simulink model "ASM_Traffic_MultiCore"  (R2026a)
settings: Solver=ode1  StartTime=SIM.tstart.v  StopTime=SIM.tend.v  FixedStep=SIM.StepSize.v
PostLoadFcn:
  | if any(exist('dsrtsu_mdlpostloadfcn', 'file') ~= 0), dsrtsu_mdlpostloadfcn('Execute', bdroot); end
  | try, asm_mdl_postloadfcn(bdroot, 'UpdateModel', 3600); catch, disp(lasterr); end,
InitFcn:
  | , if any(exist('rtifpga_mdlclblib', 'file') ~= 0), rtifpga_mdlclblib('Init', bdroot); end,
  | , if any(exist('dsmpb_private', 'file') ~= 0), dsmpb_private('dsmpb_mdlclblib', 'Init', bdroot); end,
model workspace (MAT data in the model file):
  asmReferencePath = [0 0.01 0.02 0.03 0.04 0.05 0.06 0.07 0.08 0.09 0.1 0.11 ... (350007 elements, 50001x7)]
  roadBounds : Simulink.Parameter (value not decoded)
  safetyAxes : Simulink.Parameter (value not decoded)
undefined symbols (not defined in the file): _to_, a0b2, ASM_BrakeHydraulics_DemoSystems, ASM_VehicleDynamics_DemoSystems, b98103fe8ad365046cd0, BrakeCircuit, controllerConfig, CPT, Crankshaft, DiscIntNeverNeededParam, dsmsi, FinalDriveAssembly, MDL, ModeSignals, mu, Pos_BrakePedal_Maneuver, rad, RefSignals, roadFamilyData, roadFamilyId, s_to_rpm, SIM, SoftECU, Suspension, Tire, Transmission
libraries: ASM_Traffic_lib x135, simulink x98, ASM_Utils_lib x77, ASM_VehicleDynamics_lib x70, ASM_Environment_lib x22, dsmpblib x20, dsmsilib x15, MDLD_Utils_lib x10, ASM_BrakeHydraulics_lib x3, sl_discontinuities x2
(part 9 of 65)

== system ASM_Traffic_MultiCore/AnimationInterface/ANIMATION_INTERFACE/Lane_Sensor ==
  Environment_Animation : Inport
  Bus Selector1 : BusSelector  OutputSignals=Pos_Left[x;y;z][m],Yaw_Angle_Left[deg],MarkerType_Left[],Pos_Right[x;y;z][m],Yaw_Angle_Right[deg],MarkerType_Right[]
  Enable_Data_Transfer : Constant
  LaneSensor : dsmsilib/dsmsi_simulation_data_objects_BL1  Priority=10001  parameterStr="{\"Version\":1,\"TransformInput\":false,\"EnableInput\":true,\"Objects\":[{\"Name\":\"LaneSensor_Left\",\"TypeClass\":{\"Name\":\"Transformation\",\"Class\":1,\"SignalProperty\":null,\"TransformationProperty\":{\"TransformMatrixIn\":false,\"TransformMatrixOut\":false,\"AngleInterpretation\":0,\"TransformationOrder\":0,\"RotationOrder\":0,\"TranslationAsParameter\":false,\"Translation\":\"[0 0 0]\",\"RotationAsParameter\":false,\"Rotation\":\"[0 0 0]\",\"ScalingAsParameter\":false,\"Scaling\":\"[1 1 1]\",\"ObjectsCount\":1},\"PositionAndScaleProperty\":null,\"PositionProperty\":null},\"Children\":[],\"Oid\":1},{\"Name\":\"LaneSensor_Right\",\"TypeClass\":{\"Name\":\"Transformation\",\"Class\":1,\"SignalProperty\":null,\"TransformationProperty\":{\"TransformMatrixIn\":false,\"TransformMatrixOut\":false,\"AngleInterpretation\":0,\"TransformationOrder\":0,\"RotationOrder\":0,\"TranslationAsParameter\":false,\"Translation\":\"[0 0 0]\",\"RotationAsParameter\":false,\"Rotation\":\"[0 0 0]\",\"ScalingAsParameter\":false,\"Scaling\":\"[1 1 1]\",\"ObjectsCount\":1},\"PositionAndScaleProperty\":null,\"PositionProperty\":null},\"Children\":[],\"Oid\":2}]}"  evalStr=dsmsi(gcb, 'EvalJson')  sampleTime=-1  globalBlockId=0  objectsBlockId=dsmsi(gcb, 'GetObjectBlockId')  objectsBlockGuiOpen=dsmsi(gcb, 'GetSdoGuiStatus')  dialogIsOpen=0  blockVersion=60  highPrecision=0  validNameBckp=LaneSensor
      settings: SourceProductName=dSPACE MSI Blockset
  Sensor_L_Rotation : Subsystem
  Sensor_L_Scaling : Subsystem
  Sensor_L_Translation : Subsystem
  Sensor_R_Rotation : Subsystem
  Sensor_R_Scaling : Subsystem
  Sensor_R_Translation : Subsystem
  Sw_Pitch_Angle_Offset_For_AURELION[0|1] : Constant
  wires:
  Sw_Pitch_Angle_Offset_For_AURELION[0|1]/1 -> Sensor_L_Rotation/1(Sw_Pitch_Angle_Offset), Sensor_R_Rotation/1(Sw_Pitch_Angle_Offset)
  Bus Selector1/5 -> Sensor_R_Rotation/2(In)  "<Yaw_Angle_Right[deg]>"
  Sensor_R_Rotation/1(Out) -> LaneSensor/6
  Enable_Data_Transfer/1 -> LaneSensor/1
  Sensor_R_Scaling/1(Out) -> LaneSensor/7
  Sensor_L_Scaling/1(Out) -> LaneSensor/4
  Bus Selector1/3 -> Sensor_L_Scaling/1(In)  "<MarkerType_Left[]>"
  Sensor_L_Rotation/1(Out) -> LaneSensor/3
  Bus Selector1/2 -> Sensor_L_Rotation/2(In)  "<Yaw_Angle_Left[deg]>"
  Sensor_R_Translation/1(Out) -> LaneSensor/5
  Sensor_L_Translation/1(Out) -> LaneSensor/2
  Bus Selector1/1 -> Sensor_L_Translation/1(In)  "<Pos_Left[x;y;z][m]>"
  Bus Selector1/6 -> Sensor_R_Scaling/1(In)  "<MarkerType_Right[]>"
  Bus Selector1/4 -> Sensor_R_Translation/1(In)  "<Pos_Right[x;y;z][m]>"
  Environment_Animation/1 -> Bus Selector1/1

== system ASM_Traffic_MultiCore/AnimationInterface/ANIMATION_INTERFACE/Lane_Sensor_Dynamic_Instruments ==
  Environment_Animation : Inport
  Bus Selector3 : BusSelector  OutputSignals=Network_Item_Type_Veh[],Distance_MeasPnt_Marker_Left[m],Distance_MeasPnt_Marker_Right[m],Velocity_MeasPnt_Marker_Left[m|s],Velocity_MeasPnt_Marker_Right[m|s]
  CalcLDWState : Subsystem
  Enable_Data_Transfer : Constant
  LaneSensor_Dynamic_Instruments : dsmsilib/dsmsi_simulation_data_objects_BL1  Priority=10001  parameterStr="{\"Version\":1,\"TransformInput\":false,\"EnableInput\":true,\"Objects\":[{\"Name\":\"LDWState_L[]\",\"TypeClass\":{\"Name\":\"Signal\",\"Class\":3,\"SignalProperty\":{\"Description\":null,\"Unit\":null,\"Type\":0,\"Length\":1,\"ObjectsCount\":1},\"TransformationProperty\":null,\"PositionAndScaleProperty\":null,\"PositionProperty\":null},\"Children\":[],\"Oid\":1},{\"Name\":\"LDWState_R[]\",\"TypeClass\":{\"Name\":\"Signal\",\"Class\":3,\"SignalProperty\":{\"Description\":null,\"Unit\":null,\"Type\":0,\"Length\":1,\"ObjectsCount\":1},\"TransformationProperty\":null,\"PositionAndScaleProperty\":null,\"PositionProperty\":null},\"Children\":[],\"Oid\":2},{\"Name\":\"LatDistance Left\",\"TypeClass\":{\"Name\":\"Signal\",\"Class\":3,\"SignalProperty\":{\"Description\":null,\"Unit\":\"m\",\"Type\":0,\"Length\":1,\"ObjectsCount\":1},\"TransformationProperty\":null,\"PositionAndScaleProperty\":null,\"PositionProperty\":null},\"Children\":[],\"Oid\":3},{\"Name\":\"LatDistance Right\",\"TypeClass\":{\"Name\":\"Signal\",\"Class\":3,\"SignalProperty\":{\"Description\":null,\"Unit\":\"m\",\"Type\":0,\"Length\":1,\"ObjectsCount\":1},\"TransformationProperty\":null,\"PositionAndScaleProperty\":null,\"PositionProperty\":null},\"Children\":[],\"Oid\":4},{\"Name\":\"LatVelocity Left\",\"TypeClass\":{\"Name\":\"Signal\",\"Class\":3,\"SignalProperty\":{\"Description\":null,\"Unit\":\"m/s\",\"Type\":0,\"Length\":1,\"ObjectsCount\":1},\"TransformationProperty\":null,\"PositionAndScaleProperty\":null,\"PositionProperty\":null},\"Children\":[],\"Oid\":5},{\"Name\":\"LatVelocity Right\",\"TypeClass\":{\"Name\":\"Signal\",\"Class\":3,\"SignalProperty\":{\"Description\":null,\"Unit\":\"m/s\",\"Type\":0,\"Length\":1,\"ObjectsCount\":1},\"TransformationProperty\":null,\"PositionAndScaleProperty\":null,\"PositionProperty\":null},\"Children\":[],\"Oid\":6}]}"  evalStr=dsmsi(gcb, 'EvalJson')  sampleTime=-1  globalBlockId=0  objectsBlockId=dsmsi(gcb, 'GetObjectBlockId')  objectsBlockGuiOpen=dsmsi(gcb, 'GetSdoGuiStatus')  dialogIsOpen=0  blockVersion=60  highPrecision=0  validNameBckp=LaneSensor_Dynamic_Instruments
      settings: SourceProductName=dSPACE MSI Blockset
  Selector1 : Selector  IndexOptions=Index vector (dialog)  Indices=[1]  OutputSizes=1
  Selector2 : Selector  IndexOptions=Index vector (dialog)  Indices=[2]  OutputSizes=1
  Selector3 : Selector  IndexOptions=Index vector (dialog)  Indices=[1]  OutputSizes=1
  Selector4 : Selector  IndexOptions=Index vector (dialog)  Indices=[2]  OutputSizes=1
  wires:
  Enable_Data_Transfer/1 -> LaneSensor_Dynamic_Instruments/1
  Environment_Animation/1 -> Bus Selector3/1
  Bus Selector3/3 -> Selector2/1  "<Distance_MeasPnt_Marker_Right[m]>"
  Bus Selector3/1 -> CalcLDWState/1(NetworkItemType[])  "<Network_Item_Type_Veh[]>"
  Bus Selector3/2 -> Selector1/1  "<Distance_MeasPnt_Marker_Left[m]>"
  Bus Selector3/5 -> Selector4/1  "<Velocity_MeasPnt_Marker_Right[m|s]>"
  CalcLDWState/1(LDWState_L[]) -> LaneSensor_Dynamic_Instruments/2
  Selector2/1 -> LaneSensor_Dynamic_Instruments/5, CalcLDWState/3(Dist_R[m])
  Selector1/1 -> LaneSensor_Dynamic_Instruments/4, CalcLDWState/2(Dist_L[m])
  Bus Selector3/4 -> Selector3/1  "<Velocity_MeasPnt_Marker_Left[m|s]>"
  Selector3/1 -> LaneSensor_Dynamic_Instruments/6
  Selector4/1 -> LaneSensor_Dynamic_Instruments/7
  CalcLDWState/2(LDWState_R[]) -> LaneSensor_Dynamic_Instruments/3

== system ASM_Traffic_MultiCore/AnimationInterface/ANIMATION_INTERFACE/Sensors ==
  Transform_In : Inport
  Sw_Sensor_Selector[] : Inport  Port=2
  Sw_Sensor_Animation[] : Inport  Port=3
  Environment_Animation : Inport  Port=4
  Bus Selector1 : BusSelector  OutputSignals=ObjectSensor2D_1,ObjectSensor2D_2,ObjectSensor2D_3,ObjectSensor2D_4,ObjectSensor2D_5,ObjectSensor2D_6,ObjectSensor2D_7
  Bus Selector2 : BusSelector  OutputSignals=Line_Sensor.Pos_Road_Lane_Animation_CoorSys_E,Line_Sensor.Pos_Road_Shape_Line_Animation_CoorSys_E,Line_Sensor.Pos_Road_Shape_ContObj_Animation_CoorSys_E,Line_Sensor.Pos_Junction_Border_Animation_CoorSys_E,Line_Sensor.Pos_Junction_Shape_Line_Animation_CoorSys_E,Line_Sensor.Pos_Junction_Shape_ContObj_Animation_CoorSys_E
  Bus Selector3 : BusSelector  OutputSignals=ObjectSensor3D_1,ObjectSensor3D_2,ObjectSensor3D_3
  Bus Selector4 : BusSelector  OutputSignals=TrafficSign_Sensor_Dyn
  Bus Selector5 : BusSelector  OutputSignals=ObjectSensor3D_1_RadarEffects,ObjectSensor3D_2_RadarEffects,ObjectSensor3D_3_RadarEffects
  Bus Selector6 : BusSelector  OutputSignals=ObjectSensor3D_1_CustomPoints,ObjectSensor3D_2_CustomPoints,ObjectSensor3D_3_CustomPoints
  Enable_Data_Transfer : Constant
  Line_Sensor_Junction_Border_Points : Subsystem
  Line_Sensor_Junction_Shape_ContObj_Points : Subsystem
  Line_Sensor_Junction_Shape_Line_Points : Subsystem
  Line_Sensor_Road_Lane_Points : Subsystem
  Line_Sensor_Road_Shape_ContObj_Points : Subsystem
  Line_Sensor_Road_Shape_Line_Points : Subsystem
  Multiport Switch : MultiPortSwitch  Inputs=11  SaturateOnIntegerOverflow=off  InputSameDT=off
  Object_Sensor_2D_Points : Subsystem
  Object_Sensor_3D_CustomPoints : Subsystem
  Object_Sensor_3D_Points : Subsystem
  Object_Sensor_3D_RadarEffect_Points : Subsystem
  Reshape : Reshape
  Sensor_Points : dsmsilib/dsmsi_simulation_data_objects_BL1  Priority=10001  parameterStr="{\"Version\":1,\"TransformInput\":false,\"EnableInput\":true,\"Objects\":[{\"Oid\":1,\"Name\":\"SensorPoints\",\"TypeClass\":{\"Name\":\"Transformation\",\"Class\":1,\"SignalProperty\":null,\"TransformationProperty\":{\"ObjectsCount\":60,\"TransformMatrixIn\":false,\"TransformMatrixOut\":false,\"AngleInterpretation\":0,\"TransformationOrder\":0,\"RotationOrder\":0,\"TranslationAsParameter\":false,\"Translation\":\"[0 0 0]\",\"RotationAsParameter\":true,\"Rotation\":\"[0 0 0]\",\"ScalingAsParameter\":true,\"Scaling\":\"[1 1 1]\"},\"PositionAndScaleProperty\":null,\"PositionProperty\":null},\"Children\":[]},{\"Oid\":2,\"Name\":\"SensorPoints\",\"TypeClass\":{\"Name\":\"Transformation\",\"Class\":1,\"SignalProperty\":null,\"TransformationProperty\":{\"ObjectsCount\":60,\"TransformMatrixIn\":false,\"TransformMatrixOut\":false,\"AngleInterpretation\":0,\"TransformationOrder\":0,\"RotationOrder\":0,\"TranslationAsParameter\":false,\"Translation\":\"[0 0 0]\",\"RotationAsParameter\":true,\"Rotation\":\"[0 0 0]\",\"ScalingAsParameter\":true,\"Scaling\":\"[1 1 1]\"},\"PositionAndScaleProperty\":null,\"PositionProperty\":null},\"Children\":[]},{\"Oid\":3,\"Name\":\"SensorPoints\",\"TypeClass\":{\"Name\":\"Transformation\",\"Class\":1,\"SignalProperty\":null,\"TransformationProperty\":{\"ObjectsCount\":60,\"TransformMatrixIn\":false,\"TransformMatrixOut\":false,\"AngleInterpretation\":0,\"TransformationOrder\":0,\"RotationOrder\":0,\"TranslationAsParameter\":false,\"Translation\":\"[0 0 0]\",\"RotationAsParameter\":true,\"Rotation\":\"[0 0 0]\",\"ScalingAsParameter\":true,\"Scaling\":\"[1 1 1]\"},\"PositionAndScaleProperty\":null,\"PositionProperty\":null},\"Children\":[]},{\"Oid\":4,\"Name\":\"SensorPoints\",\"TypeClass\":{\"Name\":\"Transformation\",\"Class\":1,\"SignalProperty\":null,\"TransformationProperty\":{\"ObjectsCount\":60,\"TransformMatrixIn\":false,\"TransformMatrixOut\":false,\"AngleInterpretation\":0,\"TransformationOrder\":0,\"RotationOrder\":0,\"TranslationAsParameter\":false,\"Translation\":\"[0 0 0]\",\"RotationAsParameter\":true,\"Rotation\":\"[0 0 0]\",\"ScalingAsParameter\":true,\"Scaling\":\"[1 1 1]\"},\"PositionAndScaleProperty\":null,\"PositionProperty\":null},\"Children\":[]},{\"Oid\":5,\"Name\":\"SensorPoints\",\"TypeClass\":{\"Name\":\"Transformation\",\"Class\":1,\"SignalProperty\":null,\"TransformationProperty\":{\"ObjectsCount\":60,\"TransformMatrixIn\":false,\"TransformMatrixOut\":false,\"AngleInterpretation\":0,\"TransformationOrder\":0,\"RotationOrder\":0,\"TranslationAsParameter\":false,\"Translation\":\"[0 0 0]\",\"RotationAsParameter\":true,\"Rotation\":\"[0 0 0]\",\"ScalingAsParameter\":true,\"Scaling\":\"[1 1 1]\"},\"PositionAndScaleProperty\":null,\"PositionProperty\":null},\"Children\":[]},{\"Oid\":6,\"Name\":\"SensorPoints\",\"TypeClass\":{\"Name\":\"Transformation\",\"Class\":1,\"SignalProperty\":null,\"TransformationProperty\":{\"ObjectsCount\":60,\"TransformMatrixIn\":false,\"TransformMatrixOut\":false,\"AngleInterpretation\":0,\"TransformationOrder\":0,\"RotationOrder\":0,\"TranslationAsParameter\":false,\"Translation\":\"[0 0 0]\",\"RotationAsParameter\":true,\"Rotation\":\"[0 0 0]\",\"ScalingAsParameter\":true,\"Scaling\":\"[1 1 1]\"},\"PositionAndScaleProperty\":null,\"PositionProperty\":null},\"Children\":[]},{\"Oid\":7,\"Name\":\"SensorPoints\",\"TypeClass\":{\"Name\":\"Transformation\",\"Class\":1,\"SignalProperty\":null,\"TransformationProperty\":{\"ObjectsCount\":60,\"TransformMatrixIn\":false,\"TransformMatrixOut\":false,\"AngleInterpretation\":0,\"TransformationOrder\":0,\"RotationOrder\":0,\"TranslationAsParameter\":false,\"Translation\":\"[0 0 0]\",\"RotationAsParameter\":true,\"Rotation\":\"[0 0 0]\",\"ScalingAsParameter\":true,\"Scaling\":\"[1 1 1]\"},\"PositionAndScaleProperty\":null,\"PositionProperty\":null},\"Children\":[]},{\"Oid\":8,\"Name\":\"SensorPoints\",\"TypeClass\":{\"Name\":\"Transformation\",\"Class\":1,\"SignalProperty\":null,\"TransformationProperty\":{\"ObjectsCount\":60,\"TransformMatrixIn\":false,\"TransformMatrixOut\":false,\"AngleInterpretation\":0,\"TransformationOrder\":0,\"RotationOrder\":0,\"TranslationAsParameter\":false,\"Translation\":\"[0 0 0]\",\"RotationAsParameter\":true,\"Rotation\":\"[0 0 0]\",\"ScalingAsParameter\":true,\"Scaling\":\"[1 1 1]\"},\"PositionAndScaleProperty\":null,\"PositionProperty\":null},\"Children\":[]},{\"Oid\":9,\"Name\":\"SensorPoints\",\"TypeClass\":{\"Name\":\"Transformation\",\"Class\":1,\"SignalProperty\":null,\"TransformationProperty\":{\"ObjectsCount\":60,\"TransformMatrixIn\":false,\"TransformMatrixOut\":false,\"AngleInterpretation\":0,\"TransformationOrder\":0,\"RotationOrder\":0,\"TranslationAsParameter\":false,\"Translation\":\"[0 0 0]\",\"RotationAsParameter\":true,\"Rotation\":\"[0 0 0]\",\"ScalingAsParameter\":true,\"Scaling\":\"[1 1 1]\"},\"PositionAndScaleProperty\":null,\"PositionProperty\":null},\"Children\":[]},{\"Oid\":10,\"Name\":\"SensorPoints\",\"TypeClass\":{\"Name\":\"Transformation\",\"Class\":1,\"SignalProperty\":null,\"TransformationProperty\":{\"ObjectsCount\":60,\"TransformMatrixIn\":false,\"TransformMatrixOut\":false,\"AngleInterpretation\":0,\"TransformationOrder\":0,\"RotationOrder\":0,\"TranslationAsParameter\":false,\"Translation\":\"[0 0 0]\",\"RotationAsParameter\":true,\"Rotation\":\"[0 0 0]\",\"ScalingAsParameter\":true,\"Scaling\":\"[1 1 1]\"},\"PositionAndScaleProperty\":null,\"PositionProperty\":null},\"Children\":[]},{\"Oid\":11,\"Name\":\"SensorPoints\",\"TypeClass\":{\"Name\":\"Transformation\",\"Class\":1,\"SignalProperty\":null,\"TransformationProperty\":{\"ObjectsCount\":60,\"TransformMatrixIn\":false,\"TransformMatrixOut\":false,\"AngleInterpretation\":0,\"TransformationOrder\":0,\"RotationOrder\":0,\"TranslationAsParameter\":false,\"Translation\":\"[0 0 0]\",\"RotationAsParameter\":true,\"Rotation\":\"[0 0 0]\",\"ScalingAsParameter\":true,\"Scaling\":\"[1 1 1]\"},\"PositionAndScaleProperty\":null,\"PositionProperty\":null},\"Children\":[]},{\"Oid\":12,\"Name\":\"SensorPoints\",\"TypeClass\":{\"Name\":\"Transformation\",\"Class\":1,\"SignalProperty\":null,\"TransformationProperty\":{\"ObjectsCount\":60,\"TransformMatrixIn\":false,\"TransformMatrixOut\":false,\"AngleInterpretation\":0,\"TransformationOrder\":0,\"RotationOrder\":0,\"TranslationAsParameter\":false,\"Translation\":\"[0 0 0]\",\"RotationAsParameter\":true,\"Rotation\":\"[0 0 0]\",\"ScalingAsParameter\":true,\"Scaling\":\"[1 1 1]\"},\"PositionAndScaleProperty\":null,\"PositionProperty\":null},\"Children\":[]},{\"Oid\":13,\"Name\":\"SensorPoints\",\"TypeClass\":{\"Name\":\"Transformation\",\"Class\":1,\"SignalProperty\":null,\"TransformationProperty\":{\"ObjectsCount\":60,\"TransformMatrixIn\":false,\"TransformMatrixOut\":false,\"AngleInterpretation\":0,\"TransformationOrder\":0,\"RotationOrder\":0,\"TranslationAsParameter\":false,\"Translation\":\"[0 0 0]\",\"RotationAsParameter\":true,\"Rotation\":\"[0 0 0]\",\"ScalingAsParameter\":true,\"Scaling\":\"[1 1 1]\"},\"PositionAndScaleProperty\":null,\"PositionProperty\":null},\"Children\":[]},{\"Oid\":14,\"Name\":\"SensorPoints\",\"TypeClass\":{\"Name\":\"Transformation\",\"Class\":1,\"SignalProperty\":null,\"TransformationProperty\":{\"ObjectsCount\":60,\"TransformMatrixIn\":false,\"TransformMatrixOut\":false,\"AngleInterpretation\":0,\"TransformationOrder\":0,\"RotationOrder\":0,\"TranslationAsParameter\":false,\"Translation\":\"[0 0 0]\",\"RotationAsParameter\":true,\"Rotation\":\"[0 0 0]\",\"ScalingAsParameter\":true,\"Scaling\":\"[1 1 1]\"},\"PositionAndScaleProperty\":null,\"PositionProperty\":null},\"Children\":[]},{\"Oid\":15,\"Name\":\"SensorPoints\",\"TypeClass\":{\"Name\":\"Transformation\",\"Class\":1,\"SignalProperty\":null,\"TransformationProperty\":{\"ObjectsCount\":60,\"TransformMatrixIn\":false,\"TransformMatrixOut\":false,\"AngleInterpretation\":0,\"TransformationOrder\":0,\"RotationOrder\":0,\"TranslationAsParameter\":false,\"Translation\":\"[0 0 0]\",\"RotationAsParameter\":true,\"Rotation\":\"[0 0 0]\",\"ScalingAsParameter\":true,\"Scaling\":\"[1 1 1]\"},\"PositionAndScaleProperty\":null,\"PositionProperty\":null},\"Children\":[]},{\"Oid\":16,\"Name\":\"SensorPoints\",\"TypeClass\":{\"Name\":\"Transformation\",\"Class\":1,\"SignalProperty\":null,\"TransformationProperty\":{\"ObjectsCount\":60,\"TransformMatrixIn\":false,\"TransformMatrixOut\":false,\"AngleInterpretation\":0,\"TransformationOrder\":0,\"RotationOrder\":0,\"TranslationAsParameter\":false,\"Translation\":\"[0 0 0]\",\"RotationAsParameter\":true,\"Rotation\":\"[0 0 0]\",\"ScalingAsParameter\":true,\"Scaling\":\"[1 1 1]\"},\"PositionAndScaleProperty\":null,\"PositionProperty\":null},\"Children\":[]},{\"Oid\":17,\"Name\":\"SensorPoints\",\"TypeClass\":{\"Name\":\"Transformation\",\"Class\":1,\"SignalProperty\":null,\"TransformationProperty\":{\"ObjectsCount\":60,\"TransformMatrixIn\":false,\"TransformMatrixOut\":false,\"AngleInterpretation\":0,\"TransformationOrder\":0,\"RotationOrder\":0,\"TranslationAsParameter\":false,\"Translation\":\"[0 0 0]\",\"RotationAsParameter\":true,\"Rotation\":\"[0 0 0]\",\"ScalingAsParameter\":true,\"Scaling\":\"[1 1 1]\"},\"PositionAndScaleProperty\":null,\"PositionProperty\":null},\"Children\":[]},{\"Oid\":18,\"Name\":\"SensorPoints\",\"TypeClass\":{\"Name\":\"Transformation\",\"Class\":1,\"SignalProperty\":null,\"TransformationProperty\":{\"ObjectsCount\":60,\"TransformMatrixIn\":false,\"TransformMatrixOut\":false,\"AngleInterpretation\":0,\"TransformationOrder\":0,\"RotationOrder\":0,\"TranslationAsParameter\":false,\"Translation\":\"[0 0 0]\",\"RotationAsParameter\":true,\"Rotation\":\"[0 0 0]\",\"ScalingAsParameter\":true,\"Scaling\":\"[1 1 1]\"},\"PositionAndScaleProperty\":null,\"PositionProperty\":null},\"Children\":[]},{\"Oid\":19,\"Name\":\"SensorPoints\",\"TypeClass\":{\"Name\":\"Transformation\",\"Class\":1,\"SignalProperty\":null,\"TransformationProperty\":{\"ObjectsCount\":60,\"TransformMatrixIn\":false,\"TransformMatrixOut\":false,\"AngleInterpretation\":0,\"TransformationOrder\":0,\"RotationOrder\":0,\"TranslationAsParameter\":false,\"Translation\":\"[0 0 0]\",\"RotationAsParameter\":true,\"Rotation\":\"[0 0 0]\",\"ScalingAsParameter\":true,\"Scaling\":\"[1 1 1]\"},\"PositionAndScaleProperty\":null,\"PositionProperty\":null},\"Children\":[]},{\"Oid\":20,\"Name\":\"SensorPoints\",\"TypeClass\":{\"Name\":\"Transformation\",\"Class\":1,\"SignalProperty\":null,\"TransformationProperty\":{\"ObjectsCount\":60,\"TransformMatrixIn\":false,\"TransformMatrixOut\":false,\"AngleInterpretation\":0,\"TransformationOrder\":0,\"RotationOrder\":0,\"TranslationAsParameter\":false,\"Translation\":\"[0 0 0]\",\"RotationAsParameter\":true,\"Rotation\":\"[0 0 0]\",\"ScalingAsParameter\":true,\"Scaling\":\"[1 1 1]\"},\"PositionAndScaleProperty\":null,\"PositionProperty\":null},\"Children\":[]},{\"Oid\":21,\"Name\":\"SensorPoints\",\"TypeClass\":{\"Name\":\"Transformation\",\"Class\":1,\"SignalProperty\":null,\"TransformationProperty\":{\"ObjectsCount\":60,\"TransformMatrixIn\":false,\"TransformMatrixOut\":false,\"AngleInterpretation\":0,\"TransformationOrder\":0,\"RotationOrder\":0,\"TranslationAsParameter\":false,\"Translation\":\"[0 0 0]\",\"RotationAsParameter\":true,\"Rotation\":\"[0 0 0]\",\"ScalingAsParameter\":true,\"Scaling\":\"[1 1 1]\"},\"PositionAndScaleProperty\":null,\"PositionProperty\":null},\"Children\":[]},{\"Oid\":22,\"Name\":\"SensorPoints\",\"TypeClass\":{\"Name\":\"Transformation\",\"Class\":1,\"SignalProperty\":null,\"TransformationProperty\":{\"ObjectsCount\":60,\"TransformMatrixIn\":false,\"TransformMatrixOut\":false,\"AngleInterpretation\":0,\"TransformationOrder\":0,\"RotationOrder\":0,\"TranslationAsParameter\":false,\"Translation\":\"[0 0 0]\",\"RotationAsParameter\":true,\"Rotation\":\"[0 0 0]\",\"ScalingAsParameter\":true,\"Scaling\":\"[1 1 1]\"},\"PositionAndScaleProperty\":null,\"PositionProperty\":null},\"Children\":[]},{\"Oid\":23,\"Name\":\"SensorPoints\",\"TypeClass\":{\"Name\":\"Transformation\",\"Class\":1,\"SignalProperty\":null,\"TransformationProperty\":{\"ObjectsCount\":60,\"TransformMatrixIn\":false,\"TransformMatrixOut\":false,\"AngleInterpretation\":0,\"TransformationOrder\":0,\"RotationOrder\":0,\"TranslationAsParameter\":false,\"Translation\":\"[0 0 0]\",\"RotationAsParameter\":true,\"Rotation\":\"[0 0 0]\",\"ScalingAsParameter\":true,\"Scaling\":\"[1 1 1]\"},\"PositionAndScaleProperty\":null,\"PositionProperty\":null},\"Children\":[]},{\"Oid\":24,\"Name\":\"SensorPoints\",\"TypeClass\":{\"Name\":\"Transformation\",\"Class\":1,\"SignalProperty\":null,\"TransformationProperty\":{\"ObjectsCount\":60,\"TransformMatrixIn\":false,\"TransformMatrixOut\":false,\"AngleInterpretation\":0,\"TransformationOrder\":0,\"RotationOrder\":0,\"TranslationAsParameter\":false,\"Translation\":\"[0 0 0]\",\"RotationAsParameter\":true,\"Rotation\":\"[0 0 0]\",\"ScalingAsParameter\":true,\"Scaling\":\"[1 1 1]\"},\"PositionAndScaleProperty\":null,\"PositionProperty\":null},\"Children\":[]},{\"Oid\":25,\"Name\":\"SensorPoints\",\"TypeClass\":{\"Name\":\"Transformation\",\"Class\":1,\"SignalProperty\":null,\"TransformationProperty\":{\"ObjectsCount\":60,\"TransformMatrixIn\":false,\"TransformMatrixOut\":false,\"AngleInterpretation\":0,\"TransformationOrder\":0,\"RotationOrder\":0,\"TranslationAsParameter\":false,\"Translation\":\"[0 0 0]\",\"RotationAsParameter\":true,\"Rotation\":\"[0 0 0]\",\"ScalingAsParameter\":true,\"Scaling\":\"[1 1 1]\"},\"PositionAndScaleProperty\":null,\"PositionProperty\":null},\"Children\":[]},{\"Oid\":26,\"Name\":\"SensorPoints\",\"TypeClass\":{\"Name\":\"Transformation\",\"Class\":1,\"SignalProperty\":null,\"TransformationProperty\":{\"ObjectsCount\":60,\"TransformMatrixIn\":false,\"TransformMatrixOut\":false,\"AngleInterpretation\":0,\"TransformationOrder\":0,\"RotationOrder\":0,\"TranslationAsParameter\":false,\"Translation\":\"[0 0 0]\",\"RotationAsParameter\":true,\"Rotation\":\"[0 0 0]\",\"ScalingAsParameter\":true,\"Scaling\":\"[1 1 1]\"},\"PositionAndScaleProperty\":null,\"PositionProperty\":null},\"Children\":[]},{\"Oid\":27,\"Name\":\"SensorPoints\",\"TypeClass\":{\"Name\":\"Transformation\",\"Class\":1,\"SignalProperty\":null,\"TransformationProperty\":{\"ObjectsCount\":60,\"TransformMatrixIn\":false,\"TransformMatrixOut\":false,\"AngleInterpretation\":0,\"TransformationOrder\":0,\"RotationOrder\":0,\"TranslationAsParameter\":false,\"Translation\":\"[0 0 0]\",\"RotationAsParameter\":true,\"Rotation\":\"[0 0 0]\",\"ScalingAsParameter\":true,\"Scaling\":\"[1 1 1]\"},\"PositionAndScaleProperty\":null,\"PositionProperty\":null},\"Children\":[]},{\"Oid\":28,\"Name\":\"SensorPoints\",\"TypeClass\":{\"Name\":\"Transformation\",\"Class\":1,\"SignalProperty\":null,\"TransformationProperty\":{\"ObjectsCount\":60,\"TransformMatrixIn\":false,\"TransformMatrixOut\":false,\"AngleInterpretation\":0,\"TransformationOrder\":0,\"RotationOrder\":0,\"TranslationAsParameter\":false,\"Translation\":\"[0 0 0]\",\"RotationAsParameter\":true,\"Rotation\":\"[0 0 0]\",\"ScalingAsParameter\":true,\"Scaling\":\"[1 1 1]\"},\"PositionAndScaleProperty\":null,\"PositionProperty\":null},\"Children\":[]},{\"Oid\":29,\"Name\":\"SensorPoints\",\"TypeClass\":{\"Name\":\"Transformation\",\"Class\":1,\"SignalProperty\":null,\"TransformationProperty\":{\"ObjectsCount\":60,\"TransformMatrixIn\":false,\"TransformMatrixOut\":false,\"AngleInterpretation\":0,\"TransformationOrder\":0,\"RotationOrder\":0,\"TranslationAsParameter\":false,\"Translation\":\"[0 0 0]\",\"RotationAsParameter\":true,\"Rotation\":\"[0 0 0]\",\"ScalingAsParameter\":true,\"Scaling\":\"[1 1 1]\"},\"PositionAndScaleProperty\":null,\"PositionProperty\":null},\"Children\":[]},{\"Oid\":30,\"Name\":\"SensorPoints\",\"TypeClass\":{\"Name\":\"Transformation\",\"Class\":1,\"SignalProperty\":null,\"TransformationProperty\":{\"ObjectsCount\":60,\"TransformMatrixIn\":false,\"TransformMatrixOut\":false,\"AngleInterpretation\":0,\"TransformationOrder\":0,\"RotationOrder\":0,\"TranslationAsParameter\":false,\"Translation\":\"[0 0 0]\",\"RotationAsParameter\":true,\"Rotation\":\"[0 0 0]\",\"ScalingAsParameter\":true,\"Scaling\":\"[1 1 1]\"},\"PositionAndScaleProperty\":null,\"PositionProperty\":null},\"Children\":[]},{\"Oid\":31,\"Name\":\"SensorPoints\",\"TypeClass\":{\"Name\":\"Transformation\",\"Class\":1,\"SignalProperty\":null,\"TransformationProperty\":{\"ObjectsCount\":60,\"TransformMatrixIn\":false,\"TransformMatrixOut\":false,\"AngleInterpretation\":0,\"TransformationOrder\":0,\"RotationOrder\":0,\"TranslationAsParameter\":false,\"Translation\":\"[0 0 0]\",\"RotationAsParameter\":true,\"Rotation\":\"[0 0 0]\",\"ScalingAsParameter\":true,\"Scaling\":\"[1 1 1]\"},\"PositionAndScaleProperty\":null,\"PositionProperty\":null},\"Children\":[]},{\"Oid\":32,\"Name\":\"SensorPoints\",\"TypeClass\":{\"Name\":\"Transformation\",\"Class\":1,\"SignalProperty\":null,\"TransformationProperty\":{\"ObjectsCount\":60,\"TransformMatrixIn\":false,\"TransformMatrixOut\":false,\"AngleInterpretation\":0,\"TransformationOrder\":0,\"RotationOrder\":0,\"TranslationAsParameter\":false,\"Translation\":\"[0 0 0]\",\"RotationAsParameter\":true,\"Rotation\":\"[0 0 0]\",\"ScalingAsParameter\":true,\"Scaling\":\"[1 1 1]\"},\"PositionAndScaleProperty\":null,\"PositionProperty\":null},\"Children\":[]},{\"Oid\":33,\"Name\":\"SensorPoints\",\"TypeClass\":{\"Name\":\"Transformation\",\"Class\":1,\"SignalProperty\":null,\"TransformationProperty\":{\"ObjectsCount\":60,\"TransformMatrixIn\":false,\"TransformMatrixOut\":false,\"AngleInterpretation\":0,\"TransformationOrder\":0,\"RotationOrder\":0,\"TranslationAsParameter\":false,\"Translation\":\"[0 0 0]\",\"RotationAsParameter\":true,\"Rotation\":\"[0 0 0]\",\"ScalingAsParameter\":true,\"Scaling\":\"[1 1 1]\"},\"PositionAndScaleProperty\":null,\"PositionProperty\":null},\"Children\":[]},{\"Oid\":34,\"Name\":\"SensorPoints\",\"TypeClass\":{\"Name\":\"Transformation\",\"Class\":1,\"SignalProperty\":null,\"TransformationProperty\":{\"ObjectsCount\":60,\"TransformMatrixIn\":false,\"TransformMatrixOut\":false,\"AngleInterpretation\":0,\"TransformationOrder\":0,\"RotationOrder\":0,\"TranslationAsParameter\":false,\"Translation\":\"[0 0 0]\",\"RotationAsParameter\":true,\"Rotation\":\"[0 0 0]\",\"ScalingAsParameter\":true,\"Scaling\":\"[1 1 1]\"},\"PositionAndScaleProperty\":null,\"PositionProperty\":null},\"Children\":[]},{\"Oid\":35,\"Name\":\"SensorPoints\",\"TypeClass\":{\"Name\":\"Transformation\",\"Class\":1,\"SignalProperty\":null,\"TransformationProperty\":{\"ObjectsCount\":60,\"TransformMatrixIn\":false,\"TransformMatrixOut\":false,\"AngleInterpretation\":0,\"TransformationOrder\":0,\"RotationOrder\":0,\"TranslationAsParameter\":false,\"Translation\":\"[0 0 0]\",\"RotationAsParameter\":true,\"Rotation\":\"[0 0 0]\",\"ScalingAsParameter\":true,\"Scaling\":\"[1 1 1]\"},\"PositionAndScaleProperty\":null,\"PositionProperty\":null},\"Children\":[]},{\"Oid\":36,\"Name\":\"SensorPoints\",\"TypeClass\":{\"Name\":\"Transformation\",\"Class\":1,\"SignalProperty\":null,\"TransformationProperty\":{\"ObjectsCount\":60,\"TransformMatrixIn\":false,\"TransformMatrixOut\":false,\"AngleInterpretation\":0,\"TransformationOrder\":0,\"RotationOrder\":0,\"TranslationAsParameter\":false,\"Translation\":\"[0 0 0]\",\"RotationAsParameter\":true,\"Rotation\":\"[0 0 0]\",\"ScalingAsParameter\":true,\"Scaling\":\"[1 1 1]\"},\"PositionAndScaleProperty\":null,\"PositionProperty\":null},\"Children\":[]},{\"Oid\":37,\"Name\":\"SensorPoints\",\"TypeClass\":{\"Name\":\"Transformation\",\"Class\":1,\"SignalProperty\":null,\"TransformationProperty\":{\"ObjectsCount\":60,\"TransformMatrixIn\":false,\"TransformMatrixOut\":false,\"AngleInterpretation\":0,\"TransformationOrder\":0,\"RotationOrder\":0,\"TranslationAsParameter\":false,\"Translation\":\"[0 0 0]\",\"RotationAsParameter\":true,\"Rotation\":\"[0 0 0]\",\"ScalingAsParameter\":true,\"Scaling\":\"[1 1 1]\"},\"PositionAndScaleProperty\":null,\"PositionProperty\":null},\"Children\":[]},{\"Oid\":38,\"Name\":\"SensorPoints\",\"TypeClass\":{\"Name\":\"Transformation\",\"Class\":1,\"SignalProperty\":null,\"TransformationProperty\":{\"ObjectsCount\":60,\"TransformMatrixIn\":false,\"TransformMatrixOut\":false,\"AngleInterpretation\":0,\"TransformationOrder\":0,\"RotationOrder\":0,\"TranslationAsParameter\":false,\"Translation\":\"[0 0 0]\",\"RotationAsParameter\":true,\"Rotation\":\"[0 0 0]\",\"ScalingAsParameter\":true,\"Scaling\":\"[1 1 1]\"},\"PositionAndScaleProperty\":null,\"PositionProperty\":null},\"Children\":[]},{\"Oid\":39,\"Name\":\"SensorPoints\",\"TypeClass\":{\"Name\":\"Transformation\",\"Class\":1,\"SignalProperty\":null,\"TransformationProperty\":{\"ObjectsCount\":60,\"TransformMatrixIn\":false,\"TransformMatrixOut\":false,\"AngleInterpretation\":0,\"TransformationOrder\":0,\"RotationOrder\":0,\"TranslationAsParameter\":false,\"Translation\":\"[0 0 0]\",\"RotationAsParameter\":true,\"Rotation\":\"[0 0 0]\",\"ScalingAsParameter\":true,\"Scaling\":\"[1 1 1]\"},\"PositionAndScaleProperty\":null,\"PositionProperty\":null},\"Children\":[]},{\"Oid\":40,\"Name\":\"SensorPoints\",\"TypeClass\":{\"Name\":\"Transformation\",\"Class\":1,\"SignalProperty\":null,\"TransformationProperty\":{\"ObjectsCount\":60,\"TransformMatrixIn\":false,\"TransformMatrixOut\":false,\"AngleInterpretation\":0,\"TransformationOrder\":0,\"RotationOrder\":0,\"TranslationAsParameter\":false,\"Translation\":\"[0 0 0]\",\"RotationAsParameter\":true,\"Rotation\":\"[0 0 0]\",\"ScalingAsParameter\":true,\"Scaling\":\"[1 1 1]\"},\"PositionAndScaleProperty\":null,\"PositionProperty\":null},\"Children\":[]},{\"Oid\":41,\"Name\":\"SensorPoints\",\"TypeClass\":{\"Name\":\"Transformation\",\"Class\":1,\"SignalProperty\":null,\"TransformationProperty\":{\"ObjectsCount\":60,\"TransformMatrixIn\":false,\"TransformMatrixOut\":false,\"AngleInterpretation\":0,\"TransformationOrder\":0,\"RotationOrder\":0,\"TranslationAsParameter\":false,\"Translation\":\"[0 0 0]\",\"RotationAsParameter\":true,\"Rotation\":\"[0 0 0]\",\"ScalingAsParameter\":true,\"Scaling\":\"[1 1 1]\"},\"PositionAndScaleProperty\":null,\"PositionProperty\":null},\"Children\":[]},{\"Oid\":42,\"Name\":\"SensorPoints\",\"TypeClass\":{\"Name\":\"Transformation\",\"Class\":1,\"SignalProperty\":null,\"TransformationProperty\":{\"ObjectsCount\":60,\"TransformMatrixIn\":false,\"TransformMatrixOut\":false,\"AngleInterpretation\":0,\"TransformationOrder\":0,\"RotationOrder\":0,\"TranslationAsParameter\":false,\"Translation\":\"[0 0 0]\",\"RotationAsParameter\":true,\"Rotation\":\"[0 0 0]\",\"ScalingAsParameter\":true,\"Scaling\":\"[1 1 1]\"},\"PositionAndScaleProperty\":null,\"PositionProperty\":null},\"Children\":[]},{\"Oid\":43,\"Name\":\"SensorPoints\",\"TypeClass\":{\"Name\":\"Transformation\",\"Class\":1,\"SignalProperty\":null,\"TransformationProperty\":{\"ObjectsCount\":60,\"TransformMatrixIn\":false,\"TransformMatrixOut\":false,\"AngleInterpretation\":0,\"TransformationOrder\":0,\"RotationOrder\":0,\"TranslationAsParameter\":false,\"Translation\":\"[0 0 0]\",\"RotationAsParameter\":true,\"Rotation\":\"[0 0 0]\",\"ScalingAsParameter\":true,\"Scaling\":\"[1 1 1]\"},\"PositionAndScaleProperty\":null,\"PositionProperty\":null},\"Children\":[]},{\"Oid\":44,\"Name\":\"SensorPoints\",\"TypeClass\":{\"Name\":\"Transformation\",\"Class\":1,\"SignalProperty\":null,\"TransformationProperty\":{\"ObjectsCount\":60,\"TransformMatrixIn\":false,\"TransformMatrixOut\":false,\"AngleInterpretation\":0,\"TransformationOrder\":0,\"RotationOrder\":0,\"TranslationAsParameter\":false,\"Translation\":\"[0 0 0]\",\"RotationAsParameter\":true,\"Rotation\":\"[0 0 0]\",\"ScalingAsParameter\":true,\"Scaling\":\"[1 1 1]\"},\"PositionAndScaleProperty\":null,\"PositionProperty\":null},\"Children\":[]},{\"Oid\":45,\"Name\":\"SensorPoints\",\"TypeClass\":{\"Name\":\"Transformation\",\"Class\":1,\"SignalProperty\":null,\"TransformationProperty\":{\"ObjectsCount\":60,\"TransformMatrixIn\":false,\"TransformMatrixOut\":false,\"AngleInterpretation\":0,\"TransformationOrder\":0,\"RotationOrder\":0,\"TranslationAsParameter\":false,\"Translation\":\"[0 0 0]\",\"RotationAsParameter\":true,\"Rotation\":\"[0 0 0]\",\"ScalingAsParameter\":true,\"Scaling\":\"[1 1 1]\"},\"PositionAndScaleProperty\":null,\"PositionProperty\":null},\"Children\":[]},{\"Oid\":46,\"Name\":\"SensorPoints\",\"TypeClass\":{\"Name\":\"Transformation\",\"Class\":1,\"SignalProperty\":null,\"TransformationProperty\":{\"ObjectsCount\":60,\"TransformMatrixIn\":false,\"TransformMatrixOut\":false,\"AngleInterpretation\":0,\"TransformationOrder\":0,\"RotationOrder\":0,\"TranslationAsParameter\":false,\"Translation\":\"[0 0 0]\",\"RotationAsParameter\":true,\"Rotation\":\"[0 0 0]\",\"ScalingAsParameter\":true,\"Scaling\":\"[1 1 1]\"},\"PositionAndScaleProperty\":null,\"PositionProperty\":null},\"Children\":[]},{\"Oid\":47,\"Name\":\"SensorPoints\",\"TypeClass\":{\"Name\":\"Transformation\",\"Class\":1,\"SignalProperty\":null,\"TransformationProperty\":{\"ObjectsCount\":60,\"TransformMatrixIn\":false,\"TransformMatrixOut\":false,\"AngleInterpretation\":0,\"TransformationOrder\":0,\"RotationOrder\":0,\"TranslationAsParameter\":false,\"Translation\":\"[0 0 0]\",\"RotationAsParameter\":true,\"Rotation\":\"[0 0 0]\",\"ScalingAsParameter\":true,\"Scaling\":\"[1 1 1]\"},\"PositionAndScaleProperty\":null,\"PositionProperty\":null},\"Children\":[]},{\"Oid\":48,\"Name\":\"SensorPoints\",\"TypeClass\":{\"Name\":\"Transformation\",\"Class\":1,\"SignalProperty\":null,\"TransformationProperty\":{\"ObjectsCount\":60,\"TransformMatrixIn\":false,\"TransformMatrixOut\":false,\"AngleInterpretation\":0,\"TransformationOrder\":0,\"RotationOrder\":0,\"TranslationAsParameter\":false,\"Translation\":\"[0 0 0]\",\"RotationAsParameter\":true,\"Rotation\":\"[0 0 0]\",\"ScalingAsParameter\":true,\"Scaling\":\"[1 1 1]\"},\"PositionAndScaleProperty\":null,\"PositionProperty\":null},\"Children\":[]},{\"Oid\":49,\"Name\":\"SensorPoints\",\"TypeClass\":{\"Name\":\"Transformation\",\"Class\":1,\"SignalProperty\":null,\"TransformationProperty\":{\"ObjectsCount\":60,\"TransformMatrixIn\":false,\"TransformMatrixOut\":false,\"AngleInterpretation\":0,\"TransformationOrder\":0,\"RotationOrder\":0,\"TranslationAsParameter\":false,\"Translation\":\"[0 0 0]\",\"RotationAsParameter\":true,\"Rotation\":\"[0 0 0]\",\"ScalingAsParameter\":true,\"Scaling\":\"[1 1 1]\"},\"PositionAndScaleProperty\":null,\"PositionProperty\":null},\"Children\":[]},{\"Oid\":50,\"Name\":\"SensorPoints\",\"TypeClass\":{\"Name\":\"Transformation\",\"Class\":1,\"SignalProperty\":null,\"TransformationProperty\":{\"ObjectsCount\":60,\"TransformMatrixIn\":false,\"TransformMatrixOut\":false,\"AngleInterpretation\":0,\"TransformationOrder\":0,\"RotationOrder\":0,\"TranslationAsParameter\":false,\"Translation\":\"[0 0 0]\",\"RotationAsParameter\":true,\"Rotation\":\"[0 0 0]\",\"ScalingAsParameter\":true,\"Scaling\":\"[1 1 1]\"},\"PositionAndScaleProperty\":null,\"PositionProperty\":null},\"Children\":[]},{\"Oid\":51,\"Name\":\"SensorPoints\",\"TypeClass\":{\"Name\":\"Transformation\",\"Class\":1,\"SignalProperty\":null,\"TransformationProperty\":{\"ObjectsCount\":60,\"TransformMatrixIn\":false,\"TransformMatrixOut\":false,\"AngleInterpretation\":0,\"TransformationOrder\":0,\"RotationOrder\":0,\"TranslationAsParameter\":false,\"Translation\":\"[0 0 0]\",\"RotationAsParameter\":true,\"Rotation\":\"[0 0 0]\",\"ScalingAsParameter\":true,\"Scaling\":\"[1 1 1]\"},\"PositionAndScaleProperty\":null,\"PositionProperty\":null},\"Children\":[]},{\"Oid\":52,\"Name\":\"SensorPoints\",\"TypeClass\":{\"Name\":\"Transformation\",\"Class\":1,\"SignalProperty\":null,\"TransformationProperty\":{\"ObjectsCount\":60,\"TransformMatrixIn\":false,\"TransformMatrixOut\":false,\"AngleInterpretation\":0,\"TransformationOrder\":0,\"RotationOrder\":0,\"TranslationAsParameter\":false,\"Translation\":\"[0 0 0]\",\"RotationAsParameter\":true,\"Rotation\":\"[0 0 0]\",\"ScalingAsParameter\":true,\"Scaling\":\"[1 1 1]\"},\"PositionAndScaleProperty\":null,\"PositionProperty\":null},\"Children\":[]},{\"Oid\":53,\"Name\":\"SensorPoints\",\"TypeClass\":{\"Name\":\"Transformation\",\"Class\":1,\"SignalProperty\":null,\"TransformationProperty\":{\"ObjectsCount\":60,\"TransformMatrixIn\":false,\"TransformMatrixOut\":false,\"AngleInterpretation\":0,\"TransformationOrder\":0,\"RotationOrder\":0,\"TranslationAsParameter\":false,\"Translation\":\"[0 0 0]\",\"RotationAsParameter\":true,\"Rotation\":\"[0 0 0]\",\"ScalingAsParameter\":true,\"Scaling\":\"[1 1 1]\"},\"PositionAndScaleProperty\":null,\"PositionProperty\":null},\"Children\":[]},{\"Oid\":54,\"Name\":\"SensorPoints\",\"TypeClass\":{\"Name\":\"Transformation\",\"Class\":1,\"SignalProperty\":null,\"TransformationProperty\":{\"ObjectsCount\":60,\"TransformMatrixIn\":false,\"TransformMatrixOut\":false,\"AngleInterpretation\":0,\"TransformationOrder\":0,\"RotationOrder\":0,\"TranslationAsParameter\":false,\"Translation\":\"[0 0 0]\",\"RotationAsParameter\":true,\"Rotation\":\"[0 0 0]\",\"ScalingAsParameter\":true,\"Scaling\":\"[1 1 1]\"},\"PositionAndScaleProperty\":null,\"PositionProperty\":null},\"Children\":[]},{\"Oid\":55,\"Name\":\"SensorPoints\",\"TypeClass\":{\"Name\":\"Transformation\",\"Class\":1,\"SignalProperty\":null,\"TransformationProperty\":{\"ObjectsCount\":60,\"TransformMatrixIn\":false,\"TransformMatrixOut\":false,\"AngleInterpretation\":0,\"TransformationOrder\":0,\"RotationOrder\":0,\"TranslationAsParameter\":false,\"Translation\":\"[0 0 0]\",\"RotationAsParameter\":true,\"Rotation\":\"[0 0 0]\",\"ScalingAsParameter\":true,\"Scaling\":\"[1 1 1]\"},\"PositionAndScaleProperty\":null,\"PositionProperty\":null},\"Children\":[]},{\"Oid\":56,\"Name\":\"SensorPoints\",\"TypeClass\":{\"Name\":\"Transformation\",\"Class\":1,\"SignalProperty\":null,\"TransformationProperty\":{\"ObjectsCount\":60,\"TransformMatrixIn\":false,\"TransformMatrixOut\":false,\"AngleInterpretation\":0,\"TransformationOrder\":0,\"RotationOrder\":0,\"TranslationAsParameter\":false,\"Translation\":\"[0 0 0]\",\"RotationAsParameter\":true,\"Rotation\":\"[0 0 0]\",\"ScalingAsParameter\":true,\"Scaling\":\"[1 1 1]\"},\"PositionAndScaleProperty\":null,\"PositionProperty\":null},\"Children\":[]},{\"Oid\":57,\"Name\":\"SensorPoints\",\"TypeClass\":{\"Name\":\"Transformation\",\"Class\":1,\"SignalProperty\":null,\"TransformationProperty\":{\"ObjectsCount\":60,\"TransformMatrixIn\":false,\"TransformMatrixOut\":false,\"AngleInterpretation\":0,\"TransformationOrder\":0,\"RotationOrder\":0,\"TranslationAsParameter\":false,\"Translation\":\"[0 0 0]\",\"RotationAsParameter\":true,\"Rotation\":\"[0 0 0]\",\"ScalingAsParameter\":true,\"Scaling\":\"[1 1 1]\"},\"PositionAndScaleProperty\":null,\"PositionProperty\":null},\"Children\":[]},{\"Oid\":58,\"Name\":\"SensorPoints\",\"TypeClass\":{\"Name\":\"Transformation\",\"Class\":1,\"SignalProperty\":null,\"TransformationProperty\":{\"ObjectsCount\":60,\"TransformMatrixIn\":false,\"TransformMatrixOut\":false,\"AngleInterpretation\":0,\"TransformationOrder\":0,\"RotationOrder\":0,\"TranslationAsParameter\":false,\"Translation\":\"[0 0 0]\",\"RotationAsParameter\":true,\"Rotation\":\"[0 0 0]\",\"ScalingAsParameter\":true,\"Scaling\":\"[1 1 1]\"},\"PositionAndScaleProperty\":null,\"PositionProperty\":null},\"Children\":[]},{\"Oid\":59,\"Name\":\"SensorPoints\",\"TypeClass\":{\"Name\":\"Transformation\",\"Class\":1,\"SignalProperty\":null,\"TransformationProperty\":{\"ObjectsCount\":60,\"TransformMatrixIn\":false,\"TransformMatrixOut\":false,\"AngleInterpretation\":0,\"TransformationOrder\":0,\"RotationOrder\":0,\"TranslationAsParameter\":false,\"Translation\":\"[0 0 0]\",\"RotationAsParameter\":true,\"Rotation\":\"[0 0 0]\",\"ScalingAsParameter\":true,\"Scaling\":\"[1 1 1]\"},\"PositionAndScaleProperty\":null,\"PositionProperty\":null},\"Children\":[]},{\"Oid\":60,\"Name\":\"SensorPoints\",\"TypeClass\":{\"Name\":\"Transformation\",\"Class\":1,\"SignalProperty\":null,\"TransformationProperty\":{\"ObjectsCount\":60,\"TransformMatrixIn\":false,\"TransformMatrixOut\":false,\"AngleInterpretation\":0,\"TransformationOrder\":0,\"RotationOrder\":0,\"TranslationAsParameter\":false,\"Translation\":\"[0 0 0]\",\"RotationAsParameter\":true,\"Rotation\":\"[0 0 0]\",\"ScalingAsParameter\":true,\"Scaling\":\"[1 1 1]\"},\"PositionAndScaleProperty\":null,\"PositionProperty\":null},\"Children\":[]}]}"  evalStr=dsmsi(gcb, 'EvalJson')  sampleTime=-1  globalBlockId=0  objectsBlockId=dsmsi(gcb, 'GetObjectBlockId')  objectsBlockGuiOpen=0  dialogIsOpen=0  blockVersion=60  highPrecision=0  validNameBckp=Sensor_Points
      settings: SourceProductName=dSPACE MSI Blockset
  Traffic_Sign_Sensor_Points : Subsystem
  wires:
  Multiport Switch/1 -> Reshape/1
  Enable_Data_Transfer/1 -> Sensor_Points/1
  Reshape/1 -> Sensor_Points/2
  Bus Selector2/6 -> Line_Sensor_Junction_Shape_ContObj_Points/1(ModelSignals)  "<Pos_Junction_Shape_ContObj_Animation_CoorSys_E>"
  Bus Selector2/5 -> Line_Sensor_Junction_Shape_Line_Points/1(ModelSignals)  "<Pos_Junction_Shape_Line_Animation_CoorSys_E>"
  Bus Selector2/4 -> Line_Sensor_Junction_Border_Points/1(ModelSignals)  "<Pos_Junction_Border_Animation_CoorSys_E>"
  Bus Selector2/3 -> Line_Sensor_Road_Shape_ContObj_Points/1(ModelSignals)  "<Pos_Road_Shape_ContObj_Animation_CoorSys_E>"
  Bus Selector2/2 -> Line_Sensor_Road_Shape_Line_Points/1(ModelSignals)  "<Pos_Road_Shape_Line_Animation_CoorSys_E>"
  Bus Selector2/1 -> Line_Sensor_Road_Lane_Points/1(ModelSignals)  "<Pos_Road_Lane_Animation_CoorSys_E>"
  Environment_Animation/1 -> Bus Selector4/1, Bus Selector5/1, Bus Selector6/1, Bus Selector2/1, Bus Selector1/1, Bus Selector3/1
  Bus Selector4/1 -> Traffic_Sign_Sensor_Points/1(ModelSignals)  "<TrafficSign_Sensor_Dyn>"
  Bus Selector6/1 -> Object_Sensor_3D_CustomPoints/2(ObjectSensor3D_1_CustomPoints_Animation)  "<ObjectSensor3D_1_CustomPoints>"
  Bus Selector6/3 -> Object_Sensor_3D_CustomPoints/4(ObjectSensor3D_3_CustomPoints_Animation)  "<ObjectSensor3D_3_CustomPoints>"
  Bus Selector6/2 -> Object_Sensor_3D_CustomPoints/3(ObjectSensor3D_2_CustomPoints_Animation)  "<ObjectSensor3D_2_CustomPoints>"
  Bus Selector5/3 -> Object_Sensor_3D_RadarEffect_Points/4(ObjectSensor3D_3_RadarEffects_Animation)  "<ObjectSensor3D_3_RadarEffects>"
  Bus Selector5/2 -> Object_Sensor_3D_RadarEffect_Points/3(ObjectSensor3D_2_RadarEffects_Animation)  "<ObjectSensor3D_2_RadarEffects>"
  Bus Selector5/1 -> Object_Sensor_3D_RadarEffect_Points/2(ObjectSensor3D_1_RadarEffects_Animation)  "<ObjectSensor3D_1_RadarEffects>"
  Bus Selector1/7 -> Object_Sensor_2D_Points/9(ObjectSensor2D_7_Animation)  "<ObjectSensor2D_7>"
  Bus Selector1/6 -> Object_Sensor_2D_Points/8(ObjectSensor2D_6_Animation)  "<ObjectSensor2D_6>"
  Bus Selector1/5 -> Object_Sensor_2D_Points/7(ObjectSensor2D_5_Animation)  "<ObjectSensor2D_5>"
  Bus Selector1/4 -> Object_Sensor_2D_Points/6(ObjectSensor2D_4_Animation)  "<ObjectSensor2D_4>"
  Bus Selector1/3 -> Object_Sensor_2D_Points/5(ObjectSensor2D_3_Animation)  "<ObjectSensor2D_3>"
  Bus Selector1/2 -> Object_Sensor_2D_Points/4(ObjectSensor2D_2_Animation)  "<ObjectSensor2D_2>"
  Bus Selector1/1 -> Object_Sensor_2D_Points/3(ObjectSensor2D_1_Animation)  "<ObjectSensor2D_1>"
  Sw_Sensor_Selector[]/1 -> Object_Sensor_3D_Points/1(Sw_Sensor_Selector[]), Object_Sensor_2D_Points/2(Sw_Sensor_Selector[]), Object_Sensor_3D_RadarEffect_Points/1(Sw_Sensor_Selector[]), Object_Sensor_3D_CustomPoints/1(Sw_Sensor_Selector[])
  Transform_In/1 -> Object_Sensor_2D_Points/1(Transform_In)
  Bus Selector3/3 -> Object_Sensor_3D_Points/4(ObjectSensor3D_3_Animation)  "<ObjectSensor3D_3>"
  Bus Selector3/2 -> Object_Sensor_3D_Points/3(ObjectSensor3D_2_Animation)  "<ObjectSensor3D_2>"
  Bus Selector3/1 -> Object_Sensor_3D_Points/2(ObjectSensor3D_1_Animation)  "<ObjectSensor3D_1>"
  Line_Sensor_Road_Shape_Line_Points/1(AnimationSignals) -> Multiport Switch/6
  Line_Sensor_Junction_Shape_Line_Points/1(AnimationSignals) -> Multiport Switch/9
  Line_Sensor_Junction_Shape_ContObj_Points/1(AnimationSignals) -> Multiport Switch/10
  Object_Sensor_3D_Points/1(AnimationSignals) -> Multiport Switch/2
  Traffic_Sign_Sensor_Points/1(AnimationSignals) -> Multiport Switch/4
  Object_Sensor_2D_Points/1(AnimationSignals) -> Multiport Switch/3
  Sw_Sensor_Animation[]/1 -> Multiport Switch/1
  Line_Sensor_Junction_Border_Points/1(AnimationSignals) -> Multiport Switch/8
  Line_Sensor_Road_Shape_ContObj_Points/1(AnimationSignals) -> Multiport Switch/7
  Line_Sensor_Road_Lane_Points/1(AnimationSignals) -> Multiport Switch/5
  Object_Sensor_3D_CustomPoints/1(AnimationSignals) -> Multiport Switch/12
  Object_Sensor_3D_RadarEffect_Points/1(AnimationSignals) -> Multiport Switch/11

== system ASM_Traffic_MultiCore/AnimationInterface/FcnCall/External_Samples ==
  Display : Display
      settings: Format=decimal (Stored Integer)
  dsmsi_sensor_feedback_BL1 : dsmsilib/dsmsi_sensor_feedback_BL1  Priority=10011  globalBlockStr=ASM_Traffic/AnimationInterface/ANIMATION_INTERFACE/Connection_Settings/dsmsi_connection_settings_BL1  pipeline=0  failureClass=ExposureTime  argumentLength=1  globalBlockId=dsmsi(gcb, 'GetGlobalBlockId')  sensorFailureBlockId=dsmsi(gcb, 'GetSensorFailureId')  globalUuid=7fbc0f5c-1ab5-4f7c-8d42-b98103fe8ad365046cd0-299c-42cd-a0b2-8824978edec42fda6c2b-1778-4453-86b3-4d675bee6ea0  blockVersion=60  updateFlag=1  dialogIsOpen='0'  validNameBckp=dsmsi_sensor_feedback_BL1
      settings: SourceProductName=dSPACE MSI Blockset
      settings: AttributesFormatString=|
      | Class: %<failureClass>
      | Sensor ID: %<pipeline>
  num_Samples[] : Outport
  wires:
  dsmsi_sensor_feedback_BL1/2 -> num_Samples[]/1
  dsmsi_sensor_feedback_BL1/1 -> Display/1
